simulink model "sim_openloop"  (R2024b)
settings: Solver=VariableStepAuto  StartTime=0.0  StopTime=simulation_time  RelTol=1e-3
values from neighbouring files (symbols this model uses):
  age = 18    [main_sim_openloop.m]
  height = 170    [main_sim_openloop.m]
  sampling_time = 1    [main_sim_openloop.m]
  sex = 0    [main_sim_openloop.m]
  weight = 60    [main_sim_openloop.m]
settings Model: Creator=michele.schiavo  LastModifiedBy=Michele

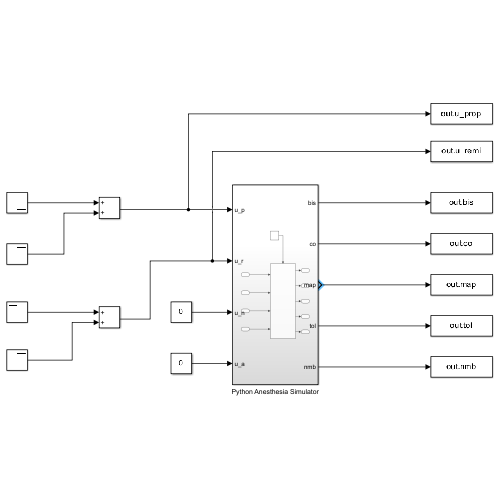
[thumbnail: Simulink's stored preview of the top-level diagram]
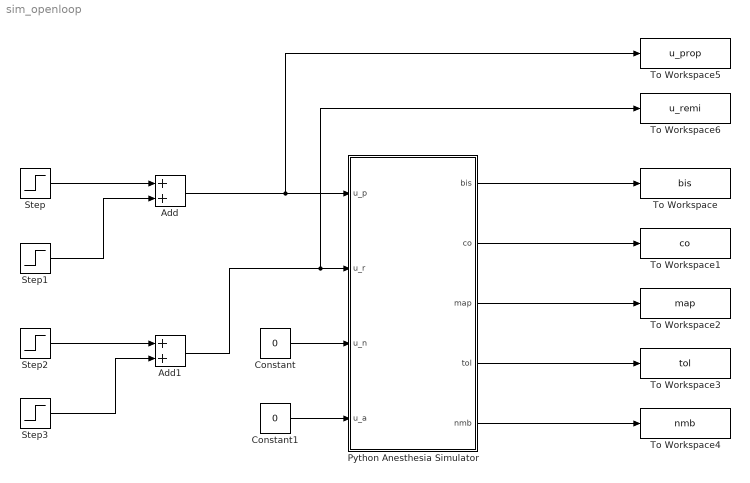
== system sim_openloop ==
  Add : Sum
  Add1 : Sum
  Constant : Constant  Value=0
  Constant1 : Constant  Value=0
  Python Anesthesia Simulator : Subsystem
  Step : Step  Time=50  Before=2  After=0  SampleTime=0
  Step1 : Step  Time=120  After=0.2  SampleTime=0
  Step2 : Step  Time=30  Before=1  After=0  SampleTime=0
  Step3 : Step  Time=120  After=0.1  SampleTime=0
  To Workspace : ToWorkspace  VariableName=bis  SaveFormat=Timeseries  SampleTime=-1
  To Workspace1 : ToWorkspace  VariableName=co  SaveFormat=Timeseries  SampleTime=-1
  To Workspace2 : ToWorkspace  VariableName=map  SaveFormat=Timeseries  SampleTime=-1
  To Workspace3 : ToWorkspace  VariableName=tol  SaveFormat=Timeseries  SampleTime=-1
  To Workspace4 : ToWorkspace  VariableName=nmb  SaveFormat=Timeseries  SampleTime=-1
  To Workspace5 : ToWorkspace  VariableName=u_prop  SaveFormat=Timeseries  SampleTime=-1
  To Workspace6 : ToWorkspace  VariableName=u_remi  SaveFormat=Timeseries  SampleTime=-1
  wires:
  Step/1 -> Add/1
  Step1/1 -> Add/2
  Step3/1 -> Add1/2
  Step2/1 -> Add1/1
  Add/1 -> To Workspace5/1, Python Anesthesia Simulator/1(u_p)
  Python Anesthesia Simulator/1(bis) -> To Workspace/1
  Add1/1 -> To Workspace6/1, Python Anesthesia Simulator/2(u_r)
  Constant/1 -> Python Anesthesia Simulator/3(u_n)
  Constant1/1 -> Python Anesthesia Simulator/4(u_a)
  Python Anesthesia Simulator/2(co) -> To Workspace1/1
  Python Anesthesia Simulator/3(map) -> To Workspace2/1
  Python Anesthesia Simulator/4(tol) -> To Workspace3/1
  Python Anesthesia Simulator/5(nmb) -> To Workspace4/1

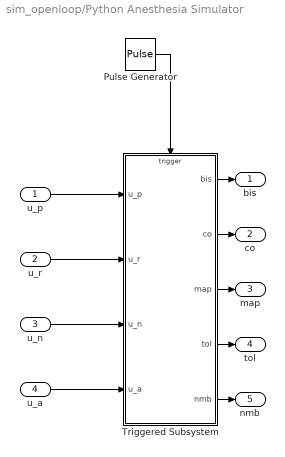
== system sim_openloop/Python Anesthesia Simulator ==
  u_p : Inport
  u_r : Inport  Port=2
  u_n : Inport  Port=3
  u_a : Inport  Port=4
  Pulse Generator : DiscretePulseGenerator  PulseType=Time based  Period=sampling_time  PulseWidth=5
  Triggered Subsystem : Subsystem  TreatAsAtomicUnit=on
  bis : Outport
  co : Outport  Port=2
  map : Outport  Port=3
  tol : Outport  Port=4
  nmb : Outport  Port=5
  wires:
  Pulse Generator/1 -> Triggered Subsystem/Trigger
  Triggered Subsystem/3(map) -> map/1
  u_p/1 -> Triggered Subsystem/1(u_p)
  Triggered Subsystem/4(tol) -> tol/1
  Triggered Subsystem/2(co) -> co/1
  Triggered Subsystem/1(bis) -> bis/1
  Triggered Subsystem/5(nmb) -> nmb/1
  u_r/1 -> Triggered Subsystem/2(u_r)
  u_n/1 -> Triggered Subsystem/3(u_n)
  u_a/1 -> Triggered Subsystem/4(u_a)

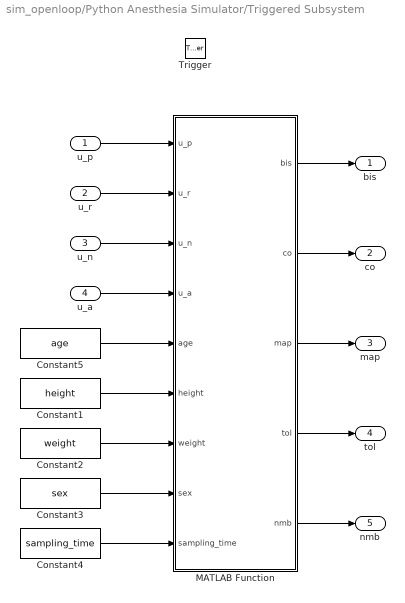
== system sim_openloop/Python Anesthesia Simulator/Triggered Subsystem ==
  u_p : Inport
  u_r : Inport  Port=2
  u_n : Inport  Port=3
  u_a : Inport  Port=4
  Trigger : TriggerPort  VariantControl=(inherit)
  Constant1 : Constant  Value=height
  Constant2 : Constant  Value=weight
  Constant3 : Constant  Value=sex
  Constant4 : Constant  Value=sampling_time
  Constant5 : Constant  Value=age
  MATLAB Function : MATLAB Function  TreatAsAtomicUnit=on
  bis : Outport
  co : Outport  Port=2
  map : Outport  Port=3
  tol : Outport  Port=4
  nmb : Outport  Port=5
  wires:
  u_p/1 -> MATLAB Function/1(u_p)
  MATLAB Function/1(bis) -> bis/1
  u_r/1 -> MATLAB Function/2(u_r)
  MATLAB Function/2(co) -> co/1
  MATLAB Function/3(map) -> map/1
  MATLAB Function/4(tol) -> tol/1
  MATLAB Function/5(nmb) -> nmb/1
  u_n/1 -> MATLAB Function/3(u_n)
  u_a/1 -> MATLAB Function/4(u_a)
  Constant5/1 -> MATLAB Function/5(age)
  Constant1/1 -> MATLAB Function/6(height)
  Constant2/1 -> MATLAB Function/7(weight)
  Constant3/1 -> MATLAB Function/8(sex)
  Constant4/1 -> MATLAB Function/9(sampling_time)

== matlab function sim_openloop/Python Anesthesia Simulator/Triggered Subsystem/MATLAB Function ==
  data: u_p input; bis output; u_r input; u_n input; u_a input; co output; map output; tol output; nmb output; age input; height input; weight input; sex input; sampling_time input
function [bis, co, map, tol, nmb] = PythonStep(u_p,u_r,u_n,u_a,age,height,weight,sex,sampling_time)
    coder.extrinsic('callPython')
    % Default value for codegen
    bis = 0; 
    co = 0;
    map = 0;
    tol = 0;
    nmb = 0;
    [bis, co, map, tol, nmb] = callPython(u_p,u_r,u_n,u_a,age,height,weight,sex,sampling_time);
end
